simulink model "MapOpt"  (R2023a)
settings: Solver=VariableStepAuto  StartTime=0.0  StopTime=10.0  RelTol=1e-3
undefined symbols (not defined in the file or in its folder): MapOpt_H_den, MapOpt_H_num, MapOpt_table, MapOpt_Ts_bp, MapOpt_Ts_ctrl, MapOpt_v_bp
settings Model: Creator=Tan_Tram  LastModifiedBy=Tan_Tram

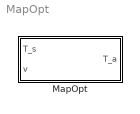
== system MapOpt ==
  MapOpt : Subsystem

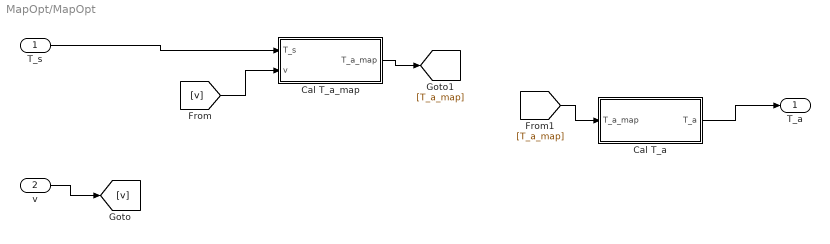
== system MapOpt/MapOpt ==
  T_s : Inport
  v : Inport  Port=2
  Cal T_a : Subsystem
  Cal T_a_map : Subsystem
  T_a : Outport
  wires:
  T_s/1 -> Cal T_a_map/1(T_s)
  v/1 -> [v]
  [v] -> Cal T_a_map/2(v)
  Cal T_a_map/1(T_a_map) -> [T_a_map]
  [T_a_map] -> Cal T_a/1(T_a_map)
  Cal T_a/1(T_a) -> T_a/1

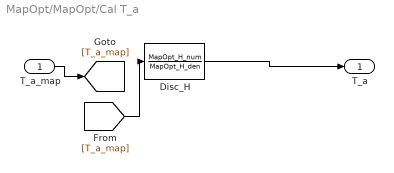
== system MapOpt/MapOpt/Cal T_a ==
  T_a_map : Inport
  Disc_H : DiscreteTransferFcn  Numerator=MapOpt_H_num  Denominator=MapOpt_H_den  SampleTime=MapOpt_Ts_ctrl
  T_a : Outport
  wires:
  T_a_map/1 -> [T_a_map]
  [T_a_map] -> Disc_H/1
  Disc_H/1 -> T_a/1

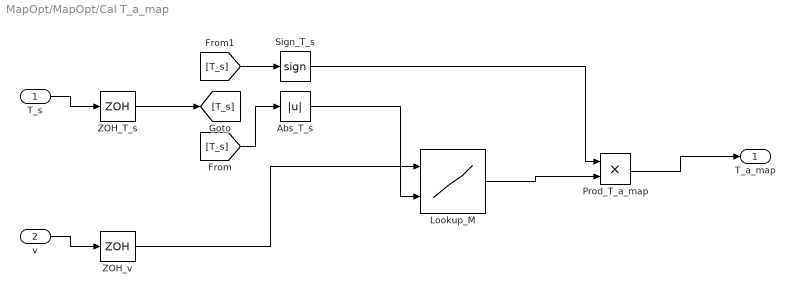
== system MapOpt/MapOpt/Cal T_a_map ==
  T_s : Inport
  v : Inport  Port=2
  Abs_T_s : Abs  SaturateOnIntegerOverflow=off
  Lookup_M : Lookup_n-D  BreakpointsForDimension1=MapOpt_v_bp  BreakpointsForDimension2=MapOpt_Ts_bp  BreakpointsForDimension3=[5, 7]  Table=MapOpt_table  ExtrapMethod=Clip  InternalRulePriority=Speed  RndMeth=Simplest
      settings: InputPortMap=u0,u1
  Prod_T_a_map : Product  Inputs=**
  Sign_T_s : Signum
  ZOH_T_s : ZeroOrderHold  SampleTime=MapOpt_Ts_ctrl
  ZOH_v : ZeroOrderHold  SampleTime=MapOpt_Ts_ctrl
  T_a_map : Outport
  wires:
  T_s/1 -> ZOH_T_s/1
  v/1 -> ZOH_v/1
  ZOH_T_s/1 -> [T_s]
  [T_s] -> Abs_T_s/1
  [T_s] -> Sign_T_s/1
  ZOH_v/1 -> Lookup_M/1
  Abs_T_s/1 -> Lookup_M/2
  Sign_T_s/1 -> Prod_T_a_map/1
  Lookup_M/1 -> Prod_T_a_map/2
  Prod_T_a_map/1 -> T_a_map/1
